simulink model "ADCS_Software_v1"  (R2026a)
settings: Solver=FixedStepAuto  StopTime=Inf  FixedStep=0.05  MaxStep=0.1
model workspace (MAT data in the model file):
  I_RW = Simulink.Parameter
  I_RW.Value = 1
  I_RW.Complexity = 'real'
  I_RW.Dimensions = [1 1]
  I_RW.CoderInfo.StorageClass = 'ExportedGlobal'
  I_RW.DataType = 'auto'
  Sig = Simulink.Signal
  Sig.Dimensions = -1
  Sig.DimensionsMode = 'auto'
  Sig.Complexity = 'auto'
  Sig.SampleTime = -1
  Sig.SamplingMode = 'auto'
  Sig.DataType = 'auto'
  h_max = Simulink.Parameter
  h_max.Value = 1.47
  h_max.Complexity = 'real'
  h_max.Dimensions = [1 1]
  h_max.DataType = 'auto'
  k_desat = Simulink.Parameter
  k_desat.Value = 1
  k_desat.Complexity = 'real'
  k_desat.Dimensions = [1 1]
  k_desat.CoderInfo.StorageClass = 'ExportedGlobal'
  k_desat.DataType = 'auto'
  kd_detumble = Simulink.Parameter
  kd_detumble.Value = 1
  kd_detumble.Complexity = 'real'
  kd_detumble.Dimensions = [1 1]
  kd_detumble.CoderInfo.StorageClass = 'ExportedGlobal'
  kd_detumble.DataType = 'auto'
  kd_hold = Simulink.Parameter
  kd_hold.Value = 1
  kd_hold.Complexity = 'real'
  kd_hold.Dimensions = [1 1]
  kd_hold.CoderInfo.StorageClass = 'ExportedGlobal'
  kd_hold.DataType = 'auto'
  kd_point = Simulink.Parameter
  kd_point.Value = 20
  kd_point.Complexity = 'real'
  kd_point.Dimensions = [1 1]
  kd_point.CoderInfo.StorageClass = 'ExportedGlobal'
  kd_point.DataType = 'auto'
  kd_slew_fast = Simulink.Parameter
  kd_slew_fast.Value = 1
  kd_slew_fast.Complexity = 'real'
  kd_slew_fast.Dimensions = [1 1]
  kd_slew_fast.CoderInfo.StorageClass = 'ExportedGlobal'
  kd_slew_fast.DataType = 'auto'
  kd_slew_slow = Simulink.Parameter
  kd_slew_slow.Value = 1
  kd_slew_slow.Complexity = 'real'
  kd_slew_slow.Dimensions = [1 1]
  kd_slew_slow.CoderInfo.StorageClass = 'ExportedGlobal'
  kd_slew_slow.DataType = 'auto'
  kd_spin = Simulink.Parameter
  kd_spin.Value = 0
  kd_spin.Complexity = 'real'
  kd_spin.Dimensions = [1 1]
  kd_spin.CoderInfo.StorageClass = 'ExportedGlobal'
  kd_spin.DataType = 'auto'
  kp_hold = Simulink.Parameter
  kp_hold.Value = 1
  kp_hold.Complexity = 'real'
  kp_hold.Dimensions = [1 1]
  kp_hold.CoderInfo.StorageClass = 'ExportedGlobal'
  kp_hold.DataType = 'auto'
  kp_point = Simulink.Parameter
  kp_point.Value = 2
  kp_point.Complexity = 'real'
  kp_point.Dimensions = [1 1]
  kp_point.CoderInfo.StorageClass = 'ExportedGlobal'
  kp_point.DataType = 'auto'
  kp_slew_fast = Simulink.Parameter
  kp_slew_fast.Value = 1
  kp_slew_fast.Complexity = 'real'
  kp_slew_fast.Dimensions = [1 1]
  kp_slew_fast.CoderInfo.StorageClass = 'ExportedGlobal'
  kp_slew_fast.DataType = 'auto'
  kp_slew_slow = Simulink.Parameter
  kp_slew_slow.Value = 1
  kp_slew_slow.Complexity = 'real'
  kp_slew_slow.Dimensions = [1 1]
  kp_slew_slow.CoderInfo.StorageClass = 'ExportedGlobal'
  kp_slew_slow.DataType = 'auto'
  kp_spin = Simulink.Parameter
  kp_spin.Value = 1
  kp_spin.Complexity = 'real'
  kp_spin.Dimensions = [1 1]
  kp_spin.CoderInfo.StorageClass = 'ExportedGlobal'
  kp_spin.DataType = 'auto'
values from neighbouring files (symbols this model uses):
  h_max = 1.47    [parameters.m]
  I_RW = 1    [parameters.m]
  k_desat = 1    [parameters.m]
  kd_detumble = 1    [parameters.m]
  kd_point = 20    [parameters.m]
  kd_spin = 0    [parameters.m]
  kp_point = 2    [parameters.m]
  kp_spin = 1    [parameters.m]
  omega_thr = 0.1    [parameters.m]
  omega_zero = 0.01    [parameters.m]
libraries: matrix_library x10, simulink x4, aerolibutil x2
(part 1 of 2)
settings Model: Creator=ADMIN  LastModifiedBy=Administrator
settings DataIOCC: ExternalInput=ds
settings RTWCC: GenerateReport=on  LaunchReport=on
settings SimscapeCC: SimscapeNominalValues="[{\"value\":\"1\",\"unit\":\"A\"},{\"value\":\"1\",\"unit\":\"bar\"},{\"value\":\"1\",\"unit\":\"cm^2\"},{\"value\":\"1\",\"unit\":\"cm^3/s\"},{\"value\":\"1\",\"unit\":\"kJ/kg\"},{\"value\":\"1\",\"unit\":\"kW\"},{\"value\":\"1\",\"unit\":\"l\"},{\"value\":\"1\",\"unit\":\"N\"},{\"value\":\"1\",\"unit\":\"N*m\"},{\"value\":\"1\",\"unit\":\"V\"}]"  SimscapeLogType=none  SimscapeLogDataHistory=5000.0

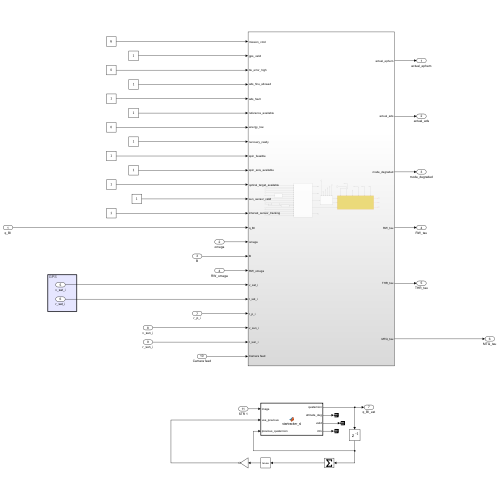
[thumbnail: Simulink's stored preview of the top-level diagram]
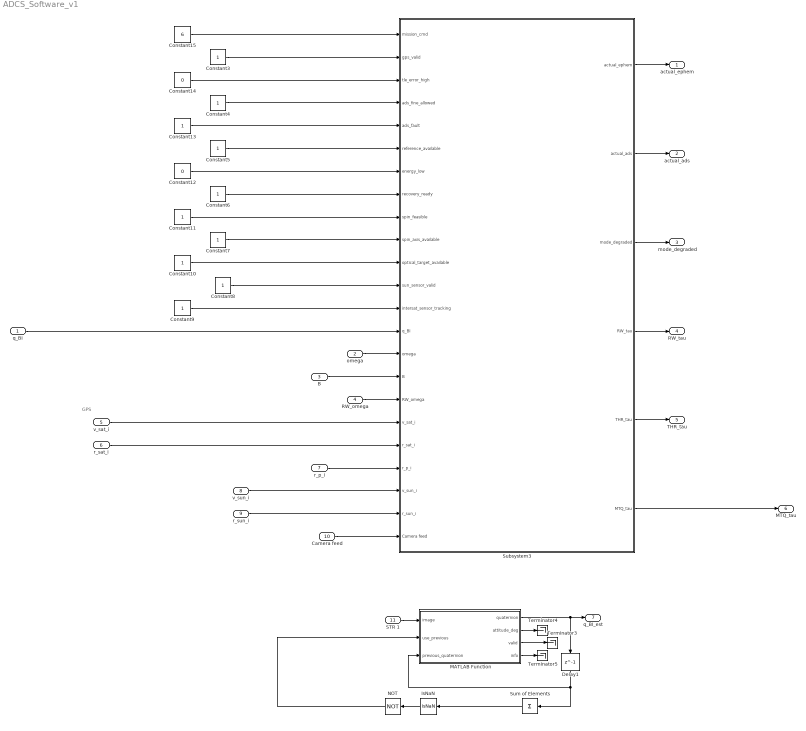
== system ADCS_Software_v1 ==
  note: GPS
  q_BI : Inport
  omega : Inport  Port=2
  B : Inport  Port=3
  RW_omega : Inport  Port=4
  v_sat_i : Inport  Port=5
  r_sat_i : Inport  Port=6
  r_p_i : Inport  Port=7
  v_sun_i : Inport  Port=8  OutDataTypeStr=double  PortDimensions=3
  r_sun_i : Inport  Port=9  OutDataTypeStr=double  PortDimensions=3
  Camera feed : Inport  Port=10  OutDataTypeStr=uint8  PortDimensions=[512,512]
  STR 1 : Inport  Port=11  OutDataTypeStr=uint8  PortDimensions=[1024,1024]
  Constant{3..11,13} (10 alike) : Constant  OutDataTypeStr=boolean
  Constant12 : Constant  Value=0  OutDataTypeStr=boolean
  Constant14 : Constant  Value=0  OutDataTypeStr=boolean
  Constant15 : Constant  Value=6  OutDataTypeStr=uint8
  Delay1 : Delay  DelayLength=1  InitialCondition=nan
  IsNaN : RelationalOperator  Operator=isNaN  OutDataTypeStr=boolean  RndMeth=Simplest  InputSameDT=off
  MATLAB Function : MATLAB Function  TreatAsAtomicUnit=on
  NOT : Logic  Operator=NOT  IconShape=distinctive  AllPortsSameDT=off  OutDataTypeStr=boolean
  Subsystem3 : Subsystem
  Sum of Elements : Sum  Inputs=+
  Terminator3 : Terminator
  Terminator4 : Terminator
  Terminator5 : Terminator
  actual_ephem : Outport
  actual_ads : Outport  Port=2
  mode_degraded : Outport  Port=3
  RW_tau : Outport  Port=4
  THR_tau : Outport  Port=5
  MTQ_tau : Outport  Port=6
  q_BI_est : Outport  Port=7  PortDimensions=[1 4]
  wires:
  Constant13/1 -> Subsystem3/5(ads_fault)
  Constant3/1 -> Subsystem3/2(gps_valid)
  Constant15/1 -> Subsystem3/1(mission_cmd)
  Constant14/1 -> Subsystem3/3(tle_error_high)
  Constant4/1 -> Subsystem3/4(ads_fine_allowed)
  Constant5/1 -> Subsystem3/6(reference_available)
  Constant12/1 -> Subsystem3/7(energy_low)
  Constant6/1 -> Subsystem3/8(recovery_ready)
  Constant10/1 -> Subsystem3/11(optical_target_available)
  Constant7/1 -> Subsystem3/10(spin_axis_available)
  Constant11/1 -> Subsystem3/9(spin_feasible)
  Constant8/1 -> Subsystem3/12(sun_sensor_valid)
  Constant9/1 -> Subsystem3/13(intersat_sensor_tracking)
  Subsystem3/1(actual_ephem) -> actual_ephem/1
  Subsystem3/2(actual_ads) -> actual_ads/1
  Subsystem3/3(mode_degraded) -> mode_degraded/1
  Subsystem3/4(RW_tau) -> RW_tau/1
  Subsystem3/5(THR_tau) -> THR_tau/1
  Subsystem3/6(MTQ_tau) -> MTQ_tau/1
  omega/1 -> Subsystem3/15(omega)
  B/1 -> Subsystem3/16(B)
  RW_omega/1 -> Subsystem3/17(RW_omega)
  v_sat_i/1 -> Subsystem3/18(v_sat_i)
  r_sat_i/1 -> Subsystem3/19(r_sat_i)
  r_p_i/1 -> Subsystem3/20(r_p_i)
  v_sun_i/1 -> Subsystem3/21(v_sun_i)
  r_sun_i/1 -> Subsystem3/22(r_sun_i)
  Camera feed/1 -> Subsystem3/23(Camera feed)
  q_BI/1 -> Subsystem3/14(q_BI)
  STR 1/1 -> MATLAB Function/1(image)
  MATLAB Function/1(quaternion) -> q_BI_est/1, Delay1/1
  MATLAB Function/4(info) -> Terminator5/1
  MATLAB Function/3(valid) -> Terminator3/1
  MATLAB Function/2(attitude_deg) -> Terminator4/1
  Sum of Elements/1 -> IsNaN/1
  IsNaN/1 -> NOT/1
  NOT/1 -> MATLAB Function/2(use_previous)
  Delay1/1 -> MATLAB Function/3(previous_quaternion), Sum of Elements/1

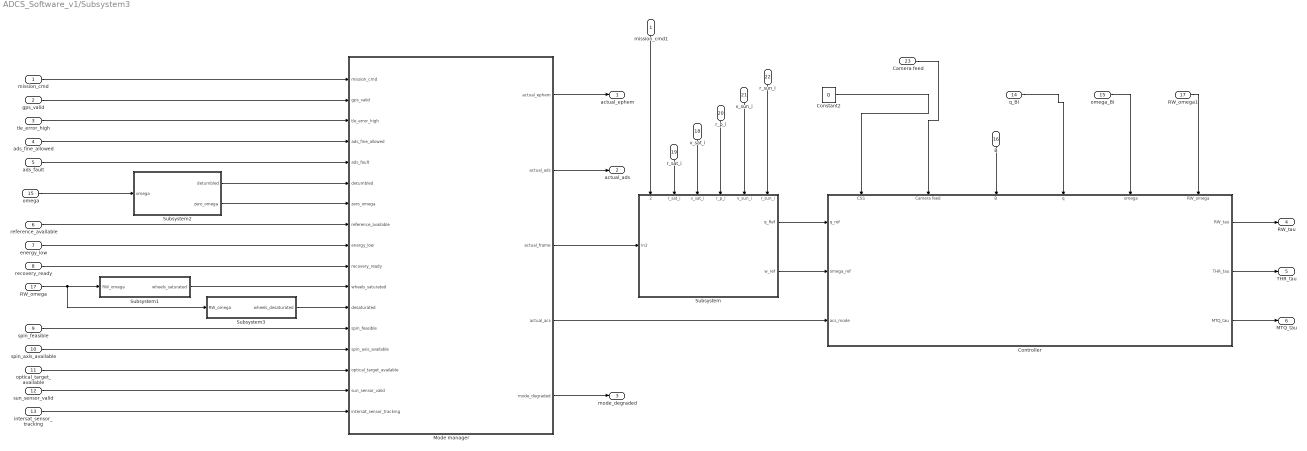
== system ADCS_Software_v1/Subsystem3 ==
  mission_cmd : Inport
  gps_valid : Inport  Port=2
  tle_error_high : Inport  Port=3
  ads_fine_allowed : Inport  Port=4
  ads_fault : Inport  Port=5
  reference_available : Inport  Port=6
  energy_low : Inport  Port=7
  recovery_ready : Inport  Port=8
  spin_feasible : Inport  Port=9
  spin_axis_available : Inport  Port=10
  optical_target_available : Inport  Port=11
  sun_sensor_valid : Inport  Port=12
  intersat_sensor_tracking : Inport  Port=13
  q_BI : Inport  Port=14
  omega : Inport  Port=15
  B : Inport  Port=16
  RW_omega : Inport  Port=17
  v_sat_i : Inport  Port=18
  r_sat_i : Inport  Port=19
  r_p_i : Inport  Port=20
  v_sun_i : Inport  Port=21
  r_sun_i : Inport  Port=22
  Camera feed : Inport  Port=23
  Constant2 : Constant  Value=0
  Controller : Subsystem
      settings: PortSchema="{\"entries\":[{\"content\":{\"sides\":[{\"content\":{\"connectorIds\":[\"In1\",\"In2\",\"In3\"]},\"type\":\"ConnectorPlacement.EquallySpacedRectSide\",\"uuid\":\"3d0ce77c-a0dd-4e63-bb58-aa259872b360\"},{\"content\":{\"connectorIds\":[\"Out1\",\"Out2\",\"Out3\"],\"side\":\"RIGHT\"},\"type\":\"ConnectorPlacement.EquallySpacedRectSide\",\"uuid\":\"c51ce6d0-00d2-499a-9be1-102c03c9909c\"},{\"content\":{\"connectorIds\":[\"In4\",\"In5\",\"In6\",\"In7\",\"In8\",\"In9\"],\"side\":\"TOP\"},\"type\":\"ConnectorPlacement.EquallySpacedRectSide\",\"uuid\":\"ed1e7bc4-2cca-4611-893f-1128994bf2d9\"},{\"content\":{\"side\":\"BOTTOM\"},\"type\":\"ConnectorPlacement.EquallySpacedRectSide\",\"uuid\":\"574e7f6a-1005-4b0c-82f8-22f1ef6841a8\"}]},\"type\":\"ConnectorPlacement.EquallySpacedConnector\",\"uuid\":\"15c446ec-b512-4968-b865-507fd68d8b0b\"}],\"packageUris\":[\"http://schema.mathworks.com/mf0/Connector/R2020b\"],\"version\":\"1.0\"}"
  Mode manager : Subsystem
  RW_omega1 : InportShadow  Port=17
  Subsystem : Subsystem
      settings: PortSchema="{\"entries\":[{\"content\":{\"sides\":[{\"content\":{\"connectorIds\":[\"In1\"]},\"type\":\"ConnectorPlacement.EquallySpacedRectSide\",\"uuid\":\"74bf1b15-53db-441c-9152-7c9ad8598452\"},{\"content\":{\"connectorIds\":[\"Out1\",\"Out2\"],\"side\":\"RIGHT\"},\"type\":\"ConnectorPlacement.EquallySpacedRectSide\",\"uuid\":\"e98e0885-3f20-4aa1-b3a1-f2c890def05c\"},{\"content\":{\"connectorIds\":[\"In2\",\"In3\",\"In4\",\"In5\",\"In6\",\"In7\"],\"side\":\"TOP\"},\"type\":\"ConnectorPlacement.EquallySpacedRectSide\",\"uuid\":\"f0898a47-7ae2-48e7-af8a-6d6327a5175a\"}]},\"type\":\"ConnectorPlacement.EquallySpacedConnector\",\"uuid\":\"b563a257-d36a-4c1e-a9df-51a9ac9caccd\"}],\"packageUris\":[\"http://schema.mathworks.com/mf0/Connector/R2020b\"],\"version\":\"1.0\"}"
  Subsystem1 : Subsystem
  Subsystem2 : Subsystem
  Subsystem3 : Subsystem
  mission_cmd1 : InportShadow
  omega_BI : InportShadow  Port=15
  actual_ephem : Outport
  actual_ads : Outport  Port=2
  mode_degraded : Outport  Port=3
  RW_tau : Outport  Port=4
  THR_tau : Outport  Port=5
  MTQ_tau : Outport  Port=6
  wires:
  spin_axis_available/1 -> Mode manager/14(spin_axis_available)
  Controller/1(RW_tau) -> RW_tau/1
  Mode manager/1(actual_ephem) -> actual_ephem/1
  Mode manager/5(mode_degraded) -> mode_degraded/1
  Constant2/1 -> Controller/4(CSS)
  gps_valid/1 -> Mode manager/2(gps_valid)
  RW_omega/1 -> Subsystem3/1(RW_omega), Subsystem1/1(RW_omega)
  Subsystem2/1(detumbled) -> Mode manager/6(detumbled)
  Mode manager/2(actual_ads) -> actual_ads/1
  tle_error_high/1 -> Mode manager/3(tle_error_high)
  Controller/3(MTQ_tau) -> MTQ_tau/1
  Mode manager/4(actual_acs) -> Controller/3(acs_mode)
  Subsystem1/1(wheels_saturated) -> Mode manager/11(wheels_saturated)
  sun_sensor_valid/1 -> Mode manager/16(sun_sensor_valid)
  recovery_ready/1 -> Mode manager/10(recovery_ready)
  Subsystem3/1(wheels_desaturated) -> Mode manager/12(desaturated)
  ads_fine_allowed/1 -> Mode manager/4(ads_fine_allowed)
  spin_feasible/1 -> Mode manager/13(spin_feasible)
  ads_fault/1 -> Mode manager/5(ads_fault)
  energy_low/1 -> Mode manager/9(energy_low)
  intersat_sensor_tracking/1 -> Mode manager/17(intersat_sensor_tracking)
  optical_target_available/1 -> Mode manager/15(optical_target_available)
  mission_cmd/1 -> Mode manager/1(mission_cmd)
  omega/1 -> Subsystem2/1(omega)
  reference_available/1 -> Mode manager/8(reference_available)
  Controller/2(THR_tau) -> THR_tau/1
  RW_omega1/1 -> Controller/9(RW_omega)
  omega_BI/1 -> Controller/8(omega)
  B/1 -> Controller/6(B)
  Mode manager/3(actual_frame) -> Subsystem/1(In2)
  Subsystem/1(q_Ref) -> Controller/1(q_ref)
  Subsystem/2(w_ref) -> Controller/2(omega_ref)
  v_sat_i/1 -> Subsystem/4(v_sat_i)
  r_sat_i/1 -> Subsystem/3(r_sat_i)
  r_p_i/1 -> Subsystem/5(r_p_i)
  v_sun_i/1 -> Subsystem/6(v_sun_i)
  r_sun_i/1 -> Subsystem/7(r_sun_i)
  Subsystem2/2(zero_omega) -> Mode manager/7(zero_omega)
  q_BI/1 -> Controller/7(q)
  Camera feed/1 -> Controller/5(Camera feed)
  mission_cmd1/1 -> Subsystem/2(mission_cmd)

== system ADCS_Software_v1/Subsystem3/Controller ==
  q_ref : Inport
  omega_ref : Inport  Port=2
  acs_mode : Inport  Port=3
  CSS : Inport  Port=4
  Camera feed : Inport  Port=5
  B : Inport  Port=6
  q : Inport  Port=7
  omega : Inport  Port=8
  RW_omega : Inport  Port=9
  Control Algorithms : Subsystem
  "error " : Subsystem
  omega1 : InportShadow  Port=8
  RW_tau : Outport
  THR_tau : Outport  Port=2
  MTQ_tau : Outport  Port=3
  wires:
  "error "/1(q_err) -> Control Algorithms/7(q_err)
  RW_omega/1 -> Control Algorithms/4(RW_omega)
  CSS/1 -> Control Algorithms/2(CSS)
  Camera feed/1 -> Control Algorithms/5(Camera feed)
  omega/1 -> Control Algorithms/3(omega)
  B/1 -> Control Algorithms/6(B)
  "error "/2(omega_err) -> Control Algorithms/8(omega_err)
  Control Algorithms/1(THR_tau) -> THR_tau/1
  Control Algorithms/2(MTQ_tau) -> MTQ_tau/1
  Control Algorithms/3(RW_tau) -> RW_tau/1
  q_ref/1 -> "error "/1(q_ref)
  q/1 -> "error "/2(q_BI)
  omega_ref/1 -> "error "/3(omega_ref)
  omega1/1 -> "error "/4(omega)
  acs_mode/1 -> Control Algorithms/1(acs_mode)

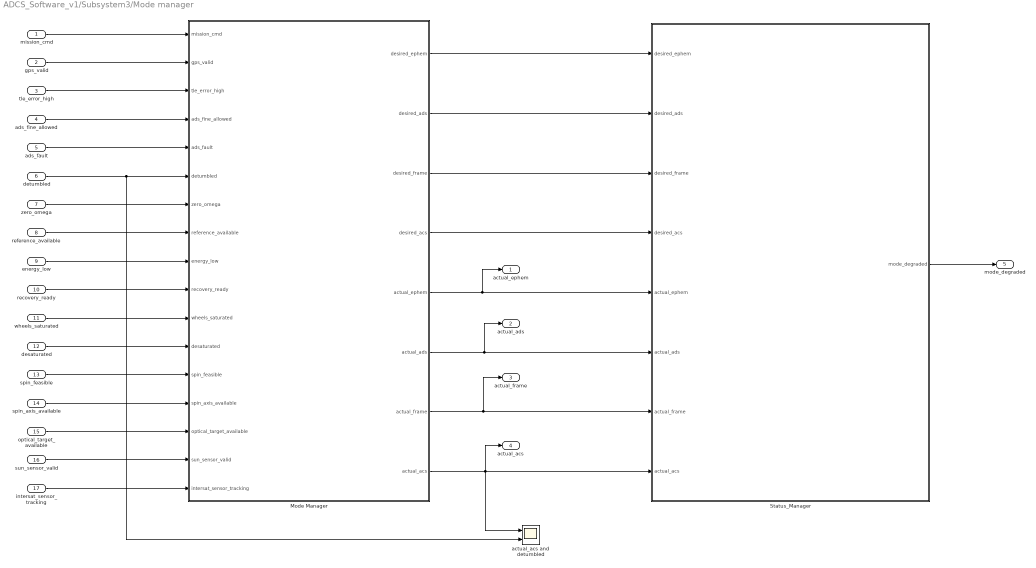
== system ADCS_Software_v1/Subsystem3/Mode manager ==
  mission_cmd : Inport
  gps_valid : Inport  Port=2
  tle_error_high : Inport  Port=3
  ads_fine_allowed : Inport  Port=4
  ads_fault : Inport  Port=5
  detumbled : Inport  Port=6
  zero_omega : Inport  Port=7
  reference_available : Inport  Port=8
  energy_low : Inport  Port=9
  recovery_ready : Inport  Port=10
  wheels_saturated : Inport  Port=11
  desaturated : Inport  Port=12
  spin_feasible : Inport  Port=13
  spin_axis_available : Inport  Port=14
  optical_target_available : Inport  Port=15
  sun_sensor_valid : Inport  Port=16
  intersat_sensor_tracking : Inport  Port=17
  Mode Manager : Subsystem
  Status_Manager : Stateflow chart  TreatAsAtomicUnit=on
  actual_acs and detumbled : Scope  NumInputPorts=2
      settings: ActiveDisplayYMinimum=-0.74999999999999978  ActiveDisplayYMaximum=6.75  DataLoggingVariableName=ScopeData3
  actual_ephem : Outport
  actual_ads : Outport  Port=2
  actual_frame : Outport  Port=3
  actual_acs : Outport  Port=4
  mode_degraded : Outport  Port=5
  wires:
  recovery_ready/1 -> Mode Manager/10(recovery_ready)
  Mode Manager/2(desired_ads) -> Status_Manager/2(desired_ads)
  Mode Manager/8(actual_acs) -> actual_acs/1, Status_Manager/8(actual_acs), actual_acs and detumbled/1
  Mode Manager/1(desired_ephem) -> Status_Manager/1(desired_ephem)
  Mode Manager/5(actual_ephem) -> actual_ephem/1, Status_Manager/5(actual_ephem)
  Mode Manager/6(actual_ads) -> actual_ads/1, Status_Manager/6(actual_ads)
  Mode Manager/7(actual_frame) -> actual_frame/1, Status_Manager/7(actual_frame)
  Mode Manager/3(desired_frame) -> Status_Manager/3(desired_frame)
  Mode Manager/4(desired_acs) -> Status_Manager/4(desired_acs)
  reference_available/1 -> Mode Manager/8(reference_available)
  mission_cmd/1 -> Mode Manager/1(mission_cmd)
  ads_fault/1 -> Mode Manager/5(ads_fault)
  ads_fine_allowed/1 -> Mode Manager/4(ads_fine_allowed)
  wheels_saturated/1 -> Mode Manager/11(wheels_saturated)
  optical_target_available/1 -> Mode Manager/15(optical_target_available)
  detumbled/1 -> Mode Manager/6(detumbled), actual_acs and detumbled/2
  intersat_sensor_tracking/1 -> Mode Manager/17(intersat_sensor_tracking)
  desaturated/1 -> Mode Manager/12(desaturated)
  spin_feasible/1 -> Mode Manager/13(spin_feasible)
  tle_error_high/1 -> Mode Manager/3(tle_error_high)
  energy_low/1 -> Mode Manager/9(energy_low)
  Status_Manager/1(mode_degraded) -> mode_degraded/1
  spin_axis_available/1 -> Mode Manager/14(spin_axis_available)
  sun_sensor_valid/1 -> Mode Manager/16(sun_sensor_valid)
  gps_valid/1 -> Mode Manager/2(gps_valid)
  zero_omega/1 -> Mode Manager/7(zero_omega)

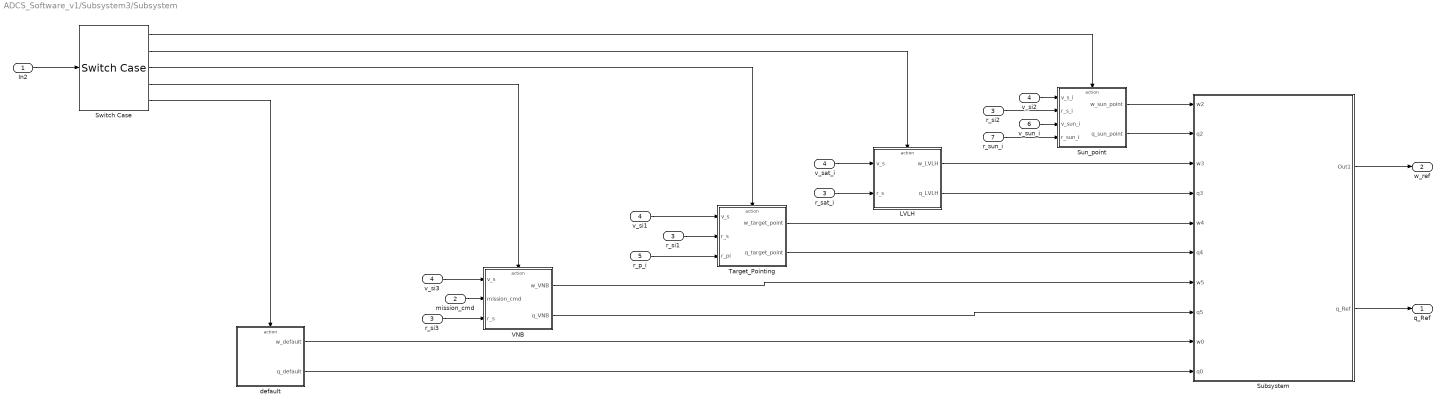
== system ADCS_Software_v1/Subsystem3/Subsystem ==
  In2 : Inport
  mission_cmd : Inport  Port=2
  r_sat_i : Inport  Port=3
  v_sat_i : Inport  Port=4
  r_p_i : Inport  Port=5
  v_sun_i : Inport  Port=6
  r_sun_i : Inport  Port=7
  LVLH : Subsystem
  Subsystem : Subsystem
  Sun_point : Subsystem
  Switch Case : SwitchCase  CaseConditions={2,3,4,5}
  Target_Pointing : Subsystem
  VNB : Subsystem
  default : Subsystem
  r_si1 : InportShadow  Port=3
  r_si2 : InportShadow  Port=3
  r_si3 : InportShadow  Port=3
  v_si1 : InportShadow  Port=4
  v_si2 : InportShadow  Port=4
  v_si3 : InportShadow  Port=4
  q_Ref : Outport
  w_ref : Outport  Port=2
  wires:
  Switch Case/5 -> default/Action
  In2/1 -> Switch Case/1
  r_si1/1 -> Target_Pointing/2(r_s)
  v_si1/1 -> Target_Pointing/1(v_s)
  LVLH/1(w_LVLH) -> Subsystem/3(w3)
  LVLH/2(q_LVLH) -> Subsystem/4(q3)
  Target_Pointing/1(w_target_point) -> Subsystem/5(w4)
  Target_Pointing/2(q_target_point) -> Subsystem/6(q4)
  default/1(w_default) -> Subsystem/9(w0)
  default/2(q_default) -> Subsystem/10(q0)
  Subsystem/1(Out1) -> w_ref/1
  v_sat_i/1 -> LVLH/1(v_s)
  r_sat_i/1 -> LVLH/2(r_s)
  v_si2/1 -> Sun_point/1(v_s_i)
  r_si2/1 -> Sun_point/2(r_s_i)
  Sun_point/1(w_sun_point) -> Subsystem/1(w2)
  Sun_point/2(q_sun_point) -> Subsystem/2(q2)
  r_p_i/1 -> Target_Pointing/3(r_pi)
  v_sun_i/1 -> Sun_point/3(v_sun_i)
  r_sun_i/1 -> Sun_point/4(r_sun_i)
  Switch Case/1 -> Sun_point/Action
  Switch Case/2 -> LVLH/Action
  Switch Case/3 -> Target_Pointing/Action
  Subsystem/2(q_Ref) -> q_Ref/1
  r_si3/1 -> VNB/3(r_s)
  v_si3/1 -> VNB/1(v_s)
  VNB/2(q_VNB) -> Subsystem/8(q5)
  VNB/1(w_VNB) -> Subsystem/7(w5)
  Switch Case/4 -> VNB/Action
  mission_cmd/1 -> VNB/2(mission_cmd)

== system ADCS_Software_v1/Subsystem3/Subsystem1 ==
  RW_omega : Inport
  Abs : Abs  SaturateOnIntegerOverflow=off
  Compare To Constant : simulink/Logic and Bit Operations/Compare To Constant  relop=>=  const=h_max*0.95  OutDataTypeStr=boolean
  Gain : Gain  Gain=I_RW
  Max of Elements : MinMax  Function=max
  wheels_saturated : Outport
  wires:
  Gain/1 -> Compare To Constant/1
  Abs/1 -> Max of Elements/1
  RW_omega/1 -> Abs/1
  Max of Elements/1 -> Gain/1
  Compare To Constant/1 -> wheels_saturated/1

== system ADCS_Software_v1/Subsystem3/Subsystem2 ==
  omega : Inport
  Compare To Constant : simulink/Logic and Bit Operations/Compare To Constant  relop=<=  const=omega_thr^2  OutDataTypeStr=boolean
  Compare To Constant1 : simulink/Logic and Bit Operations/Compare To Constant  relop=<=  const=omega_zero^2  OutDataTypeStr=boolean
  Dot Product : DotProduct  OutDataTypeStr=Inherit: Inherit via internal rule
  detumbled : Outport
  zero_omega : Outport  Port=2
  wires:
  Compare To Constant/1 -> detumbled/1
  omega/1 -> Dot Product/2, Dot Product/1
  Dot Product/1 -> Compare To Constant1/1, Compare To Constant/1
  Compare To Constant1/1 -> zero_omega/1

== system ADCS_Software_v1/Subsystem3/Subsystem3 ==
  RW_omega : Inport
  Abs : Abs  SaturateOnIntegerOverflow=off
  Compare To Constant : simulink/Logic and Bit Operations/Compare To Constant  relop=<=  const=h_max*0.25  OutDataTypeStr=boolean
  Gain : Gain  Gain=I_RW
  Max of Elements : MinMax  Function=max
  wheels_desaturated : Outport
  wires:
  Compare To Constant/1 -> wheels_desaturated/1
  Max of Elements/1 -> Gain/1
  RW_omega/1 -> Abs/1
  Abs/1 -> Max of Elements/1
  Gain/1 -> Compare To Constant/1

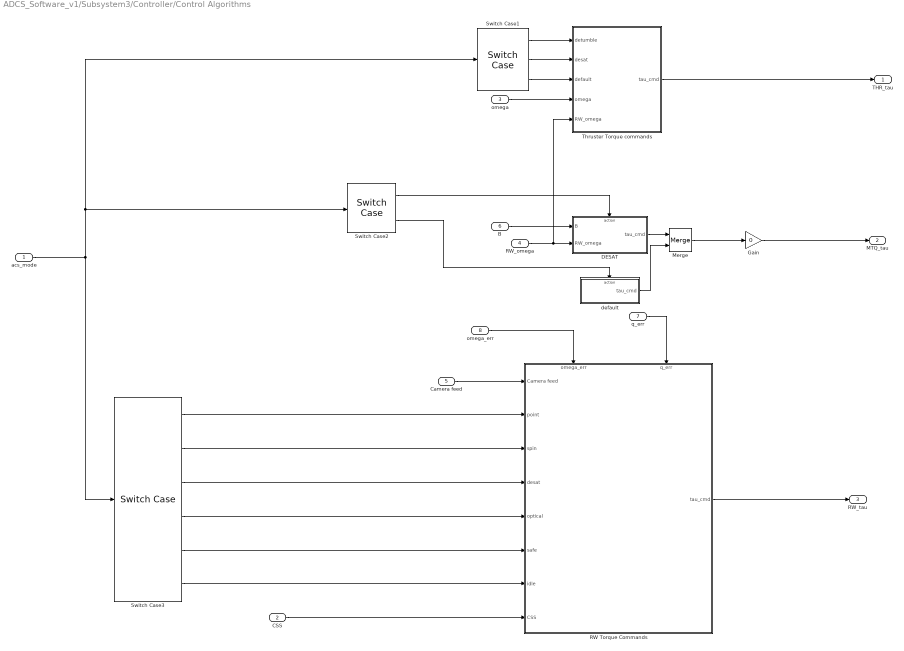
== system ADCS_Software_v1/Subsystem3/Controller/Control Algorithms ==
  acs_mode : Inport
  CSS : Inport  Port=2
  omega : Inport  Port=3
  RW_omega : Inport  Port=4
  Camera feed : Inport  Port=5
  B : Inport  Port=6
  q_err : Inport  Port=7
  omega_err : Inport  Port=8
  DESAT : Subsystem  TreatAsAtomicUnit=on
  Gain : Gain  Gain=0
  Merge : Merge
  RW Torque Commands : Subsystem
      settings: PortSchema="{\"entries\":[{\"content\":{\"sides\":[{\"content\":{\"connectorIds\":[\"In1\",\"In2\",\"In3\",\"In4\",\"In5\",\"In6\",\"In7\",\"In8\"]},\"type\":\"ConnectorPlacement.EquallySpacedRectSide\",\"uuid\":\"3d0ce77c-a0dd-4e63-bb58-aa259872b360\"},{\"content\":{\"connectorIds\":[\"Out1\"],\"side\":\"RIGHT\"},\"type\":\"ConnectorPlacement.EquallySpacedRectSide\",\"uuid\":\"c51ce6d0-00d2-499a-9be1-102c03c9909c\"},{\"content\":{\"connectorIds\":[\"In9\",\"In10\"],\"side\":\"TOP\"},\"type\":\"ConnectorPlacement.EquallySpacedRectSide\",\"uuid\":\"ed1e7bc4-2cca-4611-893f-1128994bf2d9\"}]},\"type\":\"ConnectorPlacement.EquallySpacedConnector\",\"uuid\":\"15c446ec-b512-4968-b865-507fd68d8b0b\"}],\"packageUris\":[\"http://schema.mathworks.com/mf0/Connector/R2020b\"],\"version\":\"1.0\"}"
  Switch Case1 : SwitchCase  CaseConditions={1,4}
  Switch Case2 : SwitchCase  CaseConditions={4}
  Switch Case3 : SwitchCase  CaseConditions={2,3,4,5,6}
  Thruster Torque commands : Subsystem
  default : Subsystem  TreatAsAtomicUnit=on
  THR_tau : Outport
  MTQ_tau : Outport  Port=2
  RW_tau : Outport  Port=3
  wires:
  Camera feed/1 -> RW Torque Commands/1(Camera feed)
  RW_omega/1 -> Thruster Torque commands/5(RW_omega), DESAT/2(RW_omega)
  B/1 -> DESAT/1(B)
  CSS/1 -> RW Torque Commands/8(CSS)
  omega/1 -> Thruster Torque commands/4(omega)
  omega_err/1 -> RW Torque Commands/9(omega_err)
  q_err/1 -> RW Torque Commands/10(q_err)
  Switch Case1/1 -> Thruster Torque commands/1(detumble)
  Switch Case1/3 -> Thruster Torque commands/3(default)
  default/1(tau_cmd) -> Merge/2
  Switch Case2/2 -> default/Action
  DESAT/1(tau_cmd) -> Merge/1
  Merge/1 -> Gain/1
  Switch Case2/1 -> DESAT/Action
  Switch Case3/1 -> RW Torque Commands/2(point)
  Switch Case3/2 -> RW Torque Commands/3(spin)
  Switch Case3/3 -> RW Torque Commands/4(desat)
  Switch Case3/6 -> RW Torque Commands/7(idle)
  acs_mode/1 -> Switch Case3/1, Switch Case1/1, Switch Case2/1
  Gain/1 -> MTQ_tau/1
  RW Torque Commands/1(tau_cmd) -> RW_tau/1
  Thruster Torque commands/1(tau_cmd) -> THR_tau/1
  Switch Case1/2 -> Thruster Torque commands/2(desat)
  Switch Case3/4 -> RW Torque Commands/5(optical)
  Switch Case3/5 -> RW Torque Commands/6(safe)

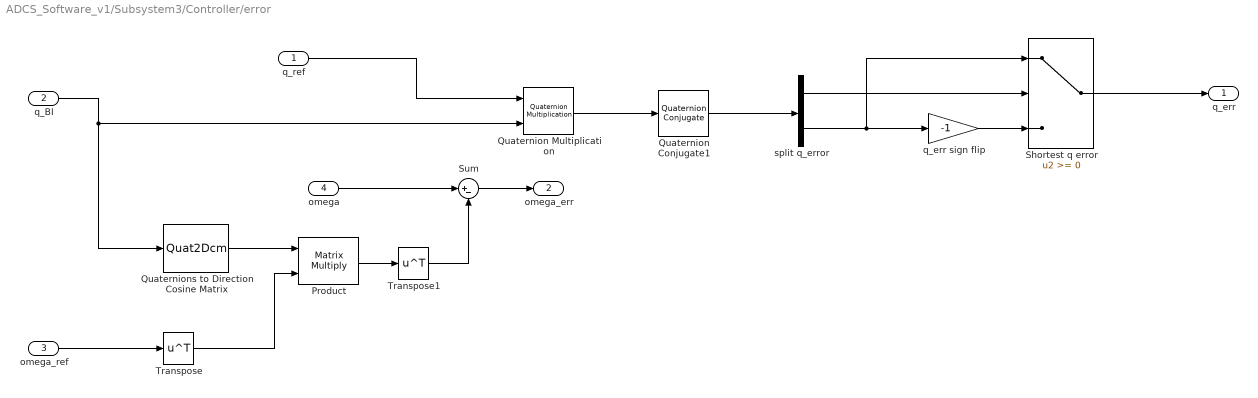
== system ADCS_Software_v1/Subsystem3/Controller/error  ==
  q_ref : Inport
  q_BI : Inport  Port=2
  omega_ref : Inport  Port=3
  omega : Inport  Port=4
  Product : Product  Multiplication=Matrix(*)
  Quaternion Conjugate1 : aerolibutil/Quaternion Conjugate
  Quaternion Multiplication : aerolibutil/Quaternion Multiplication
  Quaternions to Direction Cosine Matrix : Quat2Dcm
  Shortest q error : Switch  SaturateOnIntegerOverflow=off  InputSameDT=off
  Sum : Sum  Inputs=|+-
  Transpose : Math  Operator=transpose
  Transpose1 : Math  Operator=transpose
  q_err sign flip : Gain  Gain=-1
  split q_error : Demux  Outputs=[1 3]
  q_err : Outport
  omega_err : Outport  Port=2
  wires:
  Sum/1 -> omega_err/1
  Quaternion Multiplication/1 -> Quaternion Conjugate1/1
  q_BI/1 -> Quaternions to Direction Cosine Matrix/1, Quaternion Multiplication/2
  omega/1 -> Sum/1
  Shortest q error/1 -> q_err/1
  split q_error/2 -> Shortest q error/1, q_err sign flip/1
  split q_error/1 -> Shortest q error/2
  q_err sign flip/1 -> Shortest q error/3
  Quaternions to Direction Cosine Matrix/1 -> Product/1
  Product/1 -> Transpose1/1
  omega_ref/1 -> Transpose/1
  Transpose/1 -> Product/2
  Transpose1/1 -> Sum/2
  Quaternion Conjugate1/1 -> split q_error/1
  q_ref/1 -> Quaternion Multiplication/1

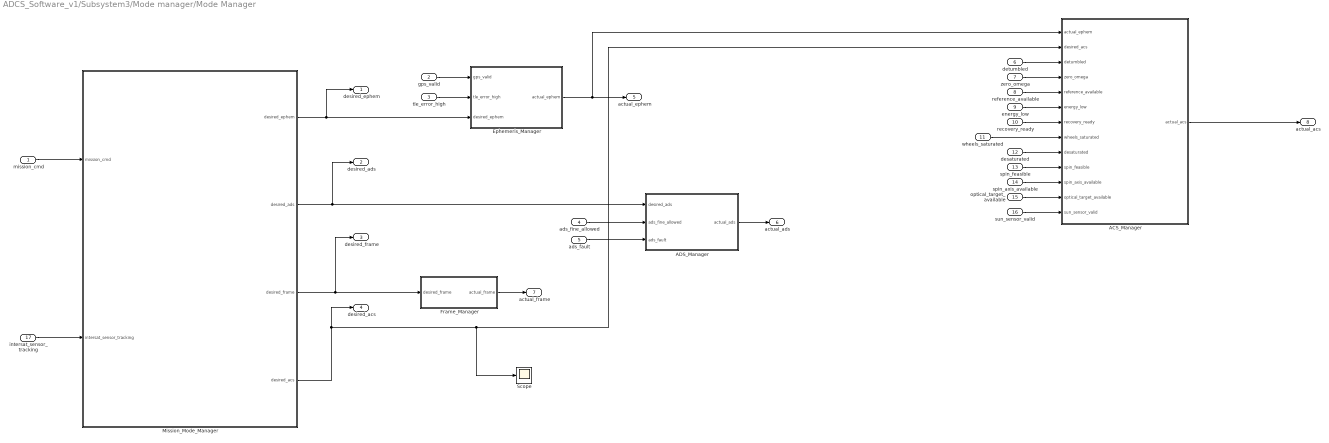
== system ADCS_Software_v1/Subsystem3/Mode manager/Mode Manager ==
  mission_cmd : Inport  OutDataTypeStr=uint8  PortDimensions=1
  gps_valid : Inport  Port=2  OutDataTypeStr=boolean  PortDimensions=1
  tle_error_high : Inport  Port=3  OutDataTypeStr=boolean  PortDimensions=1
  ads_fine_allowed : Inport  Port=4  OutDataTypeStr=boolean  PortDimensions=1
  ads_fault : Inport  Port=5  OutDataTypeStr=boolean  PortDimensions=1
  detumbled : Inport  Port=6  OutDataTypeStr=boolean  PortDimensions=1
  zero_omega : Inport  Port=7
  reference_available : Inport  Port=8  OutDataTypeStr=boolean  PortDimensions=1
  energy_low : Inport  Port=9  OutDataTypeStr=boolean  PortDimensions=1
  recovery_ready : Inport  Port=10  OutDataTypeStr=boolean  PortDimensions=1
  wheels_saturated : Inport  Port=11  OutDataTypeStr=boolean  PortDimensions=1
  desaturated : Inport  Port=12  OutDataTypeStr=boolean  PortDimensions=1
  spin_feasible : Inport  Port=13  OutDataTypeStr=boolean  PortDimensions=1
  spin_axis_available : Inport  Port=14  OutDataTypeStr=boolean  PortDimensions=1
  optical_target_available : Inport  Port=15  OutDataTypeStr=boolean  PortDimensions=1
  sun_sensor_valid : Inport  Port=16  OutDataTypeStr=boolean  PortDimensions=1
  intersat_sensor_tracking : Inport  Port=17  OutDataTypeStr=boolean  PortDimensions=1
  ACS_Manager : Stateflow chart  TreatAsAtomicUnit=on
      settings: PortSchema="{\"entries\":[{\"content\":{\"sides\":[{\"content\":{\"connectorIds\":[\"In2\",\"In1\",\"In3\",\"In4\",\"In5\",\"In6\",\"In7\",\"In8\",\"In9\",\"In10\",\"In11\",\"In12\",\"In13\"]},\"type\":\"ConnectorPlacement.EquallySpacedRectSide\",\"uuid\":\"c64f5ed7-7a07-4761-a251-d625087249f8\"},{\"content\":{\"connectorIds\":[\"Out1\"],\"side\":\"RIGHT\"},\"type\":\"ConnectorPlacement.EquallySpacedRectSide\",\"uuid\":\"ff17dfa7-5a32-4799-bec0-131df3b46d45\"},{\"content\":{\"side\":\"TOP\"},\"type\":\"ConnectorPlacement.EquallySpacedRectSide\",\"uuid\":\"acaf274e-12ec-4fab-ab7e-ad580afcef6e\"},{\"content\":{\"side\":\"BOTTOM\"},\"type\":\"ConnectorPlacement.EquallySpacedRectSide\",\"uuid\":\"23b8eb5a-32b2-43f2-9f21-5c184446e61f\"}]},\"type\":\"ConnectorPlacement.EquallySpacedConnector\",\"uuid\":\"7d19de63-b993-417e-b6e9-9dc888da130b\"}],\"packageUris\":[\"http://schema.mathworks.com/mf0/Connector/R2020b\"],\"version\":\"1.0\"}"
  ADS_Manager : Stateflow chart  TreatAsAtomicUnit=on
  Ephemeris_Manager : Stateflow chart  TreatAsAtomicUnit=on
      settings: PortSchema="{\"entries\":[{\"content\":{\"sides\":[{\"content\":{\"connectorIds\":[\"In2\",\"In3\",\"In1\"]},\"type\":\"ConnectorPlacement.EquallySpacedRectSide\",\"uuid\":\"cbbccf67-8c60-498d-a98a-76db8747fb3a\"},{\"content\":{\"connectorIds\":[\"Out1\"],\"side\":\"RIGHT\"},\"type\":\"ConnectorPlacement.EquallySpacedRectSide\",\"uuid\":\"743b35d2-d398-4833-9c20-93b5e77612f2\"},{\"content\":{\"side\":\"TOP\"},\"type\":\"ConnectorPlacement.EquallySpacedRectSide\",\"uuid\":\"56075cc1-c683-438a-85bf-78d94186ffa6\"}]},\"type\":\"ConnectorPlacement.EquallySpacedConnector\",\"uuid\":\"bae867d4-09fc-4097-a23b-eff5fb3633ac\"}],\"packageUris\":[\"http://schema.mathworks.com/mf0/Connector/R2020b\"],\"version\":\"1.0\"}"
  Frame_Manager : Stateflow chart  TreatAsAtomicUnit=on
  Mission_Mode_Manager : Stateflow chart  TreatAsAtomicUnit=on
  Scope : Scope
      settings: ActiveDisplayYMinimum=-1  ActiveDisplayYMaximum=1  DataLoggingVariableName=ScopeData4
  desired_ephem : Outport
  desired_ads : Outport  Port=2
  desired_frame : Outport  Port=3
  desired_acs : Outport  Port=4
  actual_ephem : Outport  Port=5
  actual_ads : Outport  Port=6
  actual_frame : Outport  Port=7
  actual_acs : Outport  Port=8
  wires:
  sun_sensor_valid/1 -> ACS_Manager/13(sun_sensor_valid)
  ACS_Manager/1(actual_acs) -> actual_acs/1
  Mission_Mode_Manager/4(desired_acs) -> Scope/1, ACS_Manager/1(desired_acs), desired_acs/1
  energy_low/1 -> ACS_Manager/6(energy_low)
  Mission_Mode_Manager/1(desired_ephem) -> Ephemeris_Manager/1(desired_ephem), desired_ephem/1
  Frame_Manager/1(actual_frame) -> actual_frame/1
  optical_target_available/1 -> ACS_Manager/12(optical_target_available)
  Mission_Mode_Manager/2(desired_ads) -> desired_ads/1, ADS_Manager/1(desired_ads)
  tle_error_high/1 -> Ephemeris_Manager/3(tle_error_high)
  reference_available/1 -> ACS_Manager/5(reference_available)
  detumbled/1 -> ACS_Manager/3(detumbled)
  wheels_saturated/1 -> ACS_Manager/8(wheels_saturated)
  Mission_Mode_Manager/3(desired_frame) -> desired_frame/1, Frame_Manager/1(desired_frame)
  ADS_Manager/1(actual_ads) -> actual_ads/1
  ads_fine_allowed/1 -> ADS_Manager/2(ads_fine_allowed)
  Ephemeris_Manager/1(actual_ephem) -> actual_ephem/1, ACS_Manager/2(actual_ephem)
  gps_valid/1 -> Ephemeris_Manager/2(gps_valid)
  intersat_sensor_tracking/1 -> Mission_Mode_Manager/2(intersat_sensor_tracking)
  ads_fault/1 -> ADS_Manager/3(ads_fault)
  recovery_ready/1 -> ACS_Manager/7(recovery_ready)
  mission_cmd/1 -> Mission_Mode_Manager/1(mission_cmd)
  spin_axis_available/1 -> ACS_Manager/11(spin_axis_available)
  desaturated/1 -> ACS_Manager/9(desaturated)
  spin_feasible/1 -> ACS_Manager/10(spin_feasible)
  zero_omega/1 -> ACS_Manager/4(zero_omega)

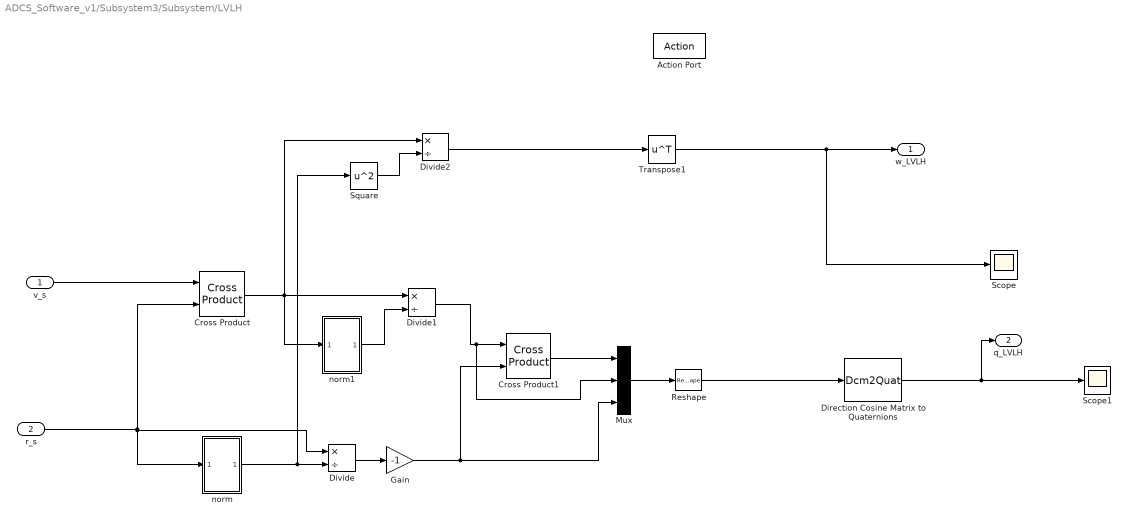
== system ADCS_Software_v1/Subsystem3/Subsystem/LVLH ==
  v_s : Inport
  r_s : Inport  Port=2
  Action Port : ActionPort  ActionPortLabel=case [ 3 ]:
  Cross Product : matrix_library/Cross Product
  Cross Product1 : matrix_library/Cross Product
  Direction Cosine Matrix to Quaternions : Dcm2Quat
  Divide : Product  Inputs=*/
  Divide1 : Product  Inputs=*/
  Divide2 : Product  Inputs=*/
  Gain : Gain  Gain=-1
  Mux : Mux  Inputs=3
  Reshape : Reshape  OutputDimensionality=Customize  OutputDimensions=[3,3]
  Scope : Scope
      settings: ActiveDisplayYMinimum=-1  ActiveDisplayYMaximum=1  DataLoggingVariableName=ScopeData6
  Scope1 : Scope
      settings: ActiveDisplayYMinimum=-0.82867069291103368  ActiveDisplayYMaximum=0.87774872275294546
  Square : Math  Operator=square
  Transpose1 : Math  Operator=transpose
  norm : Subsystem
  norm1 : Subsystem
  w_LVLH : Outport
  q_LVLH : Outport  Port=2
  wires:
  Transpose1/1 -> Scope/1, w_LVLH/1
  Divide/1 -> Gain/1
  Divide1/1 -> Mux/2, Cross Product1/1
  norm1/1(Out1) -> Divide1/2
  Cross Product1/1 -> Mux/1
  Mux/1 -> Reshape/1
  Square/1 -> Divide2/2
  v_s/1 -> Cross Product/1
  r_s/1 -> norm/1(In1), Divide/1, Cross Product/2
  norm/1(Out1) -> Square/1, Divide/2
  Divide2/1 -> Transpose1/1
  Direction Cosine Matrix to Quaternions/1 -> q_LVLH/1, Scope1/1
  Gain/1 -> Mux/3, Cross Product1/2
  Cross Product/1 -> Divide2/1, Divide1/1, norm1/1(In1)
  Reshape/1 -> Direction Cosine Matrix to Quaternions/1

== system ADCS_Software_v1/Subsystem3/Subsystem/Subsystem ==
  w2 : Inport
  q2 : Inport  Port=2
  w3 : Inport  Port=3
  q3 : Inport  Port=4
  w4 : Inport  Port=5
  q4 : Inport  Port=6
  w5 : Inport  Port=7
  q5 : Inport  Port=8
  w0 : Inport  Port=9
  q0 : Inport  Port=10
  Merge : Merge  Inputs=5
  Merge1 : Merge  Inputs=5
  Transpose2 : Math  Operator=transpose
  Out1 : Outport
  q_Ref : Outport  Port=2
  wires:
  q4/1 -> Merge1/3
  q3/1 -> Merge1/2
  Merge/1 -> Transpose2/1
  q2/1 -> Merge1/1
  Merge1/1 -> q_Ref/1
  w4/1 -> Merge/3
  w3/1 -> Merge/2
  w2/1 -> Merge/1
  Transpose2/1 -> Out1/1
  q0/1 -> Merge1/5
  q5/1 -> Merge1/4
  w0/1 -> Merge/5
  w5/1 -> Merge/4

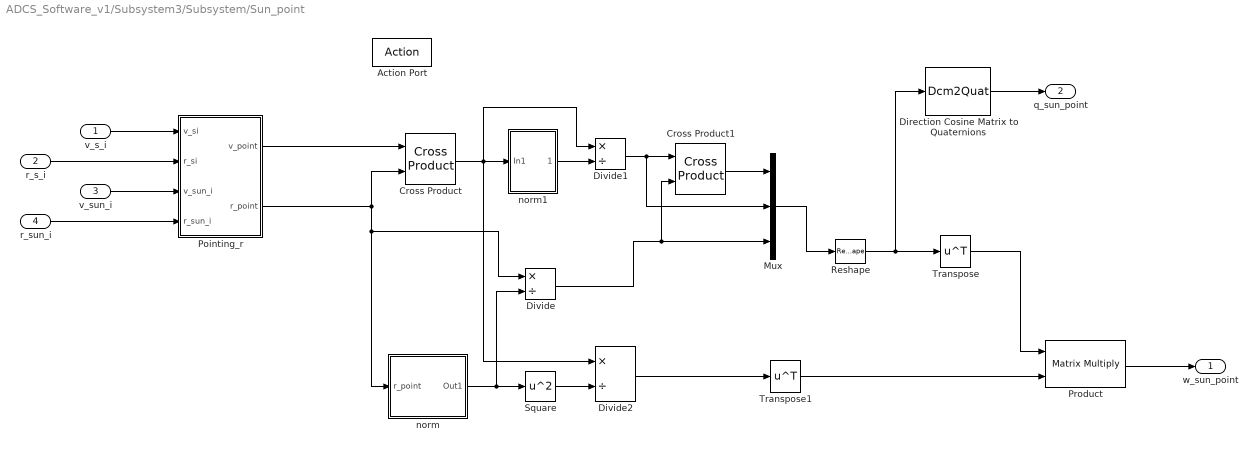
== system ADCS_Software_v1/Subsystem3/Subsystem/Sun_point ==
  v_s_i : Inport
  r_s_i : Inport  Port=2
  v_sun_i : Inport  Port=3
  r_sun_i : Inport  Port=4
  Action Port : ActionPort  ActionPortLabel=case [ 2 ]:
  Cross Product : matrix_library/Cross Product
  Cross Product1 : matrix_library/Cross Product
  Direction Cosine Matrix to Quaternions : Dcm2Quat
  Divide : Product  Inputs=*/
  Divide1 : Product  Inputs=*/
  Divide2 : Product  Inputs=*/
  Mux : Mux  Inputs=3
  Pointing_r : Subsystem
  Product : Product  Multiplication=Matrix(*)
  Reshape : Reshape  OutputDimensionality=Customize  OutputDimensions=[3,3]
  Square : Math  Operator=square
  Transpose : Math  Operator=transpose
  Transpose1 : Math  Operator=transpose
  norm : Subsystem
  norm1 : Subsystem
  w_sun_point : Outport
  q_sun_point : Outport  Port=2
  wires:
  Product/1 -> w_sun_point/1
  Direction Cosine Matrix to Quaternions/1 -> q_sun_point/1
  Transpose/1 -> Product/1
  Reshape/1 -> Transpose/1, Direction Cosine Matrix to Quaternions/1
  Transpose1/1 -> Product/2
  Cross Product1/1 -> Mux/1
  Divide/1 -> Cross Product1/2, Mux/3
  Square/1 -> Divide2/2
  norm1/1(Out1) -> Divide1/2
  Divide1/1 -> Mux/2, Cross Product1/1
  Cross Product/1 -> norm1/1(In1), Divide1/1, Divide2/1
  Pointing_r/2(r_point) -> Divide/1, norm/1(r_point), Cross Product/2
  Mux/1 -> Reshape/1
  norm/1(Out1) -> Square/1, Divide/2
  Divide2/1 -> Transpose1/1
  Pointing_r/1(v_point) -> Cross Product/1
  r_s_i/1 -> Pointing_r/2(r_si)
  v_s_i/1 -> Pointing_r/1(v_si)
  v_sun_i/1 -> Pointing_r/3(v_sun_i)
  r_sun_i/1 -> Pointing_r/4(r_sun_i)

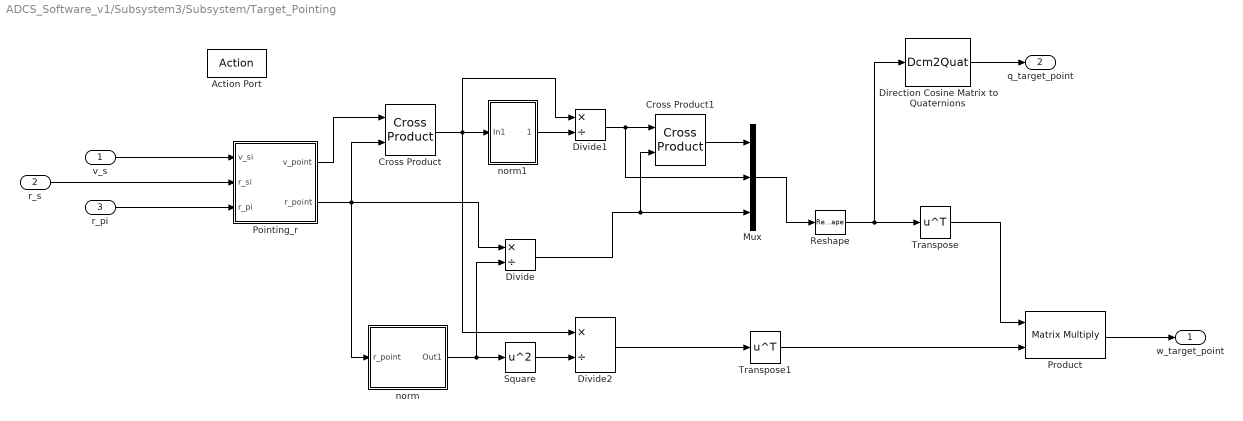
== system ADCS_Software_v1/Subsystem3/Subsystem/Target_Pointing ==
  v_s : Inport
  r_s : Inport  Port=2
  r_pi : Inport  Port=3
  Action Port : ActionPort  ActionPortLabel=case [ 4 ]:
  Cross Product : matrix_library/Cross Product
  Cross Product1 : matrix_library/Cross Product
  Direction Cosine Matrix to Quaternions : Dcm2Quat
  Divide : Product  Inputs=*/
  Divide1 : Product  Inputs=*/
  Divide2 : Product  Inputs=*/
  Mux : Mux  Inputs=3
  Pointing_r : Subsystem
  Product : Product  Multiplication=Matrix(*)
  Reshape : Reshape  OutputDimensionality=Customize  OutputDimensions=[3,3]
  Square : Math  Operator=square
  Transpose : Math  Operator=transpose
  Transpose1 : Math  Operator=transpose
  norm : Subsystem
  norm1 : Subsystem
  w_target_point : Outport
  q_target_point : Outport  Port=2
  wires:
  v_s/1 -> Pointing_r/1(v_si)
  r_s/1 -> Pointing_r/2(r_si)
  Pointing_r/1(v_point) -> Cross Product/1
  Divide2/1 -> Transpose1/1
  norm/1(Out1) -> Divide/2, Square/1
  Mux/1 -> Reshape/1
  Pointing_r/2(r_point) -> norm/1(r_point), Divide/1, Cross Product/2
  Cross Product/1 -> Divide2/1, Divide1/1, norm1/1(In1)
  Divide1/1 -> Cross Product1/1, Mux/2
  norm1/1(Out1) -> Divide1/2
  Square/1 -> Divide2/2
  Divide/1 -> Mux/3, Cross Product1/2
  Cross Product1/1 -> Mux/1
  Transpose1/1 -> Product/2
  Reshape/1 -> Direction Cosine Matrix to Quaternions/1, Transpose/1
  Transpose/1 -> Product/1
  Direction Cosine Matrix to Quaternions/1 -> q_target_point/1
  Product/1 -> w_target_point/1
  r_pi/1 -> Pointing_r/3(r_pi)

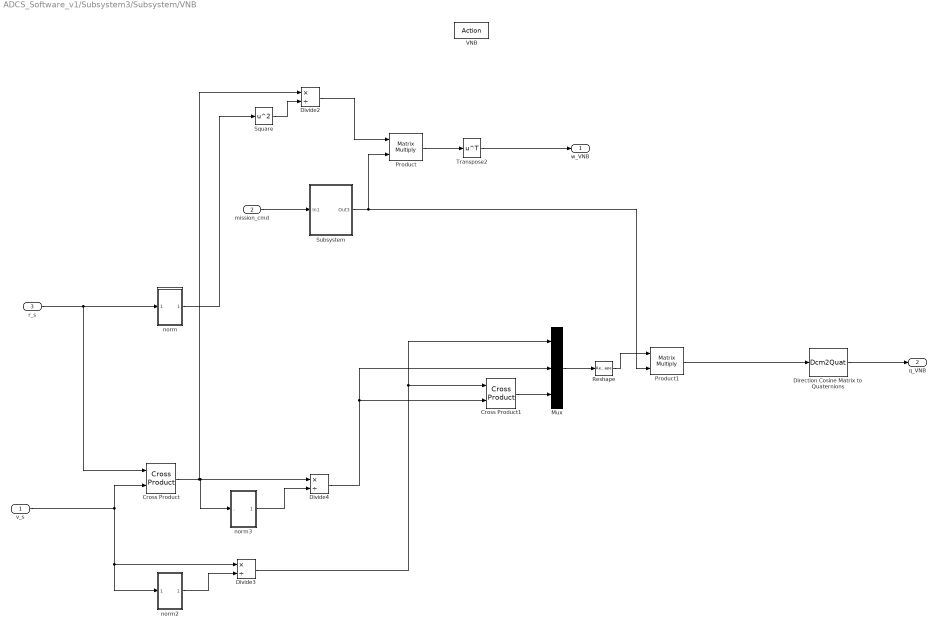
== system ADCS_Software_v1/Subsystem3/Subsystem/VNB ==
  v_s : Inport
  mission_cmd : Inport  Port=2
  r_s : Inport  Port=3
  VNB : ActionPort  ActionPortLabel=case [ 5 ]:
  Cross Product : matrix_library/Cross Product
  Cross Product1 : matrix_library/Cross Product
  Direction Cosine Matrix to Quaternions : Dcm2Quat
  Divide2 : Product  Inputs=*/
  Divide3 : Product  Inputs=*/
  Divide4 : Product  Inputs=*/
  Mux : Mux  Inputs=3
  Product : Product  Multiplication=Matrix(*)
  Product1 : Product  Multiplication=Matrix(*)
  Reshape : Reshape  OutputDimensionality=Customize  OutputDimensions=[3,3]
  Square : Math  Operator=square
  Subsystem : Subsystem
  Transpose2 : Math  Operator=transpose
  norm : Subsystem
  norm2 : Subsystem
  norm3 : Subsystem
  w_VNB : Outport
  q_VNB : Outport  Port=2
  wires:
  Product/1 -> Transpose2/1
  Square/1 -> Divide2/2
  r_s/1 -> norm/1(In1), Cross Product/1
  norm/1(Out1) -> Square/1
  Direction Cosine Matrix to Quaternions/1 -> q_VNB/1
  Product1/1 -> Direction Cosine Matrix to Quaternions/1
  norm2/1(Out1) -> Divide3/2
  v_s/1 -> Divide3/1, norm2/1(v_s), Cross Product/2
  Divide3/1 -> Mux/1, Cross Product1/1
  Cross Product/1 -> Divide2/1, norm3/1(,), Divide4/1
  norm3/1(Out1) -> Divide4/2
  Divide4/1 -> Cross Product1/2, Mux/2
  Cross Product1/1 -> Mux/3
  mission_cmd/1 -> Subsystem/1(In1)
  Subsystem/1(Out3) -> Product/2, Product1/2
  Mux/1 -> Reshape/1
  Reshape/1 -> Product1/1
  Transpose2/1 -> w_VNB/1
  Divide2/1 -> Product/1

== system ADCS_Software_v1/Subsystem3/Subsystem/default ==
  Action Port : ActionPort  ActionPortLabel=default:
  Constant : Constant  Value=[0; 0; 0]
  Constant1 : Constant  Value=[1 0 0 0]
  w_default : Outport
  q_default : Outport  Port=2
  wires:
  Constant1/1 -> q_default/1
  Constant/1 -> w_default/1

== system ADCS_Software_v1/Subsystem3/Controller/Control Algorithms/DESAT ==
  B : Inport
  RW_omega : Inport  Port=2
  desat : ActionPort  ActionPortLabel=case [ 4 ]:
  Cross Product : matrix_library/Cross Product
  Divide : Product  Inputs=*/
  Dot Product : DotProduct  OutDataTypeStr=Inherit: Inherit via internal rule
  Gain : Gain  Gain=-k_desat
  tau_cmd : Outport
  wires:
  B/1 -> Dot Product/1, Dot Product/2, Cross Product/2
  Divide/1 -> Gain/1
  Gain/1 -> tau_cmd/1
  Cross Product/1 -> Divide/1
  RW_omega/1 -> Cross Product/1
  Dot Product/1 -> Divide/2

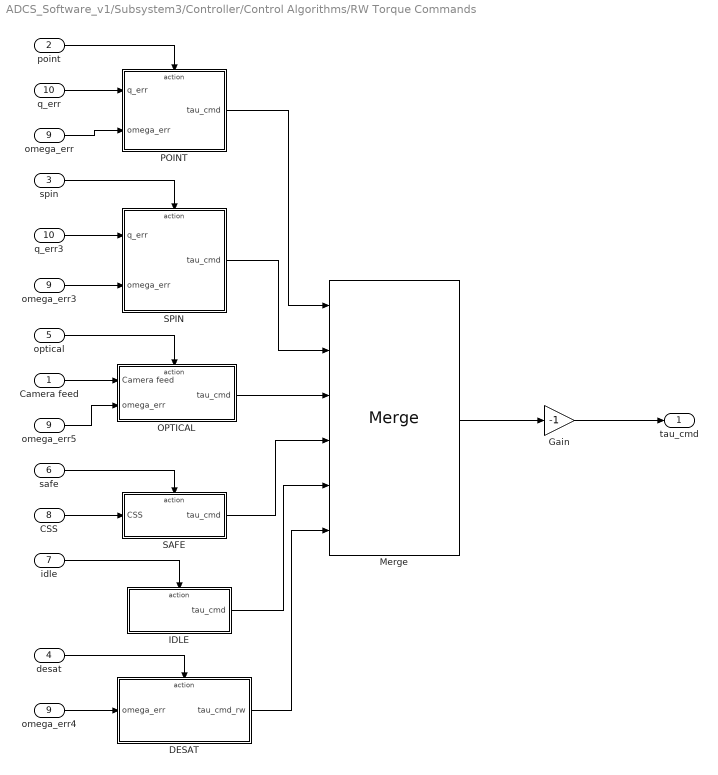
== system ADCS_Software_v1/Subsystem3/Controller/Control Algorithms/RW Torque Commands ==
  Camera feed : Inport
  point : Inport  Port=2
  spin : Inport  Port=3
  desat : Inport  Port=4
  optical : Inport  Port=5
  safe : Inport  Port=6
  idle : Inport  Port=7
  CSS : Inport  Port=8
  omega_err : Inport  Port=9
  q_err : Inport  Port=10
  DESAT : Subsystem  TreatAsAtomicUnit=on
  Gain : Gain  Gain=-1
  IDLE : Subsystem  TreatAsAtomicUnit=on
  Merge : Merge  Inputs=6
  OPTICAL : Subsystem  TreatAsAtomicUnit=on
  POINT : Subsystem  TreatAsAtomicUnit=on
  SAFE : Subsystem  TreatAsAtomicUnit=on
  SPIN : Subsystem  TreatAsAtomicUnit=on
  omega_err3 : InportShadow  Port=9
  omega_err4 : InportShadow  Port=9
  omega_err5 : InportShadow  Port=9
  q_err3 : InportShadow  Port=10
  tau_cmd : Outport
  wires:
  idle/1 -> IDLE/Action
  spin/1 -> SPIN/Action
  Camera feed/1 -> OPTICAL/1(Camera feed)
  omega_err4/1 -> DESAT/1(omega_err)
  omega_err/1 -> POINT/2(omega_err)
  optical/1 -> OPTICAL/Action
  desat/1 -> DESAT/Action
  CSS/1 -> SAFE/1(CSS)
  point/1 -> POINT/Action
  omega_err3/1 -> SPIN/2(omega_err)
  safe/1 -> SAFE/Action
  q_err/1 -> POINT/1(q_err)
  q_err3/1 -> SPIN/1(q_err)
  omega_err5/1 -> OPTICAL/2(omega_err)
  POINT/1(tau_cmd) -> Merge/1
  SPIN/1(tau_cmd) -> Merge/2
  OPTICAL/1(tau_cmd) -> Merge/3
  SAFE/1(tau_cmd) -> Merge/4
  IDLE/1(tau_cmd) -> Merge/5
  DESAT/1(tau_cmd_rw) -> Merge/6
  Merge/1 -> Gain/1
  Gain/1 -> tau_cmd/1

== system ADCS_Software_v1/Subsystem3/Controller/Control Algorithms/Thruster Torque commands ==
  detumble : Inport
  desat : Inport  Port=2
  default : Inport  Port=3
  omega : Inport  Port=4
  RW_omega : Inport  Port=5
  DEFAULT : Subsystem  TreatAsAtomicUnit=on
  DESAT : Subsystem  TreatAsAtomicUnit=on
  DETUMBLE : Subsystem  TreatAsAtomicUnit=on
  Merge1 : Merge  Inputs=3
  tau_cmd : Outport
  wires:
  omega/1 -> DETUMBLE/1(omega)
  DETUMBLE/1(tau_cmd) -> Merge1/1
  Merge1/1 -> tau_cmd/1
  detumble/1 -> DETUMBLE/Action
  default/1 -> DEFAULT/Action
  DEFAULT/1(tau_cmd) -> Merge1/3
  RW_omega/1 -> DESAT/1(RW_omega)
  desat/1 -> DESAT/Action
  DESAT/1(tau_cmd) -> Merge1/2

== system ADCS_Software_v1/Subsystem3/Controller/Control Algorithms/default ==
  detumble : ActionPort  ActionPortLabel=default:
  Constant : Constant  Value=[0 0 0]
  tau_cmd : Outport
  wires:
  Constant/1 -> tau_cmd/1

== system ADCS_Software_v1/Subsystem3/Subsystem/LVLH/norm ==
  In1 : Inport
  Sqrt : Sqrt
  Square : Math  Operator=square
  Sum of Elements : Sum  Inputs=+
  Out1 : Outport
  wires:
  In1/1 -> Square/1
  Square/1 -> Sum of Elements/1
  Sum of Elements/1 -> Sqrt/1
  Sqrt/1 -> Out1/1

== system ADCS_Software_v1/Subsystem3/Subsystem/LVLH/norm1 ==
  In1 : Inport
  Sqrt : Sqrt
  Square : Math  Operator=square
  Sum of Elements : Sum  Inputs=+
  Out1 : Outport
  wires:
  Sqrt/1 -> Out1/1
  Sum of Elements/1 -> Sqrt/1
  Square/1 -> Sum of Elements/1
  In1/1 -> Square/1

== system ADCS_Software_v1/Subsystem3/Subsystem/Sun_point/Pointing_r ==
  v_si : Inport
  r_si : Inport  Port=2
  v_sun_i : Inport  Port=3
  r_sun_i : Inport  Port=4
  Sum : Sum  Inputs=|-+
  Sum1 : Sum  Inputs=|-+
  v_point : Outport
  r_point : Outport  Port=2
  wires:
  Sum1/1 -> v_point/1
  v_si/1 -> Sum1/1
  Sum/1 -> r_point/1
  r_si/1 -> Sum/1
  v_sun_i/1 -> Sum1/2
  r_sun_i/1 -> Sum/2

== system ADCS_Software_v1/Subsystem3/Subsystem/Sun_point/norm ==
  r_point : Inport
  Sqrt : Sqrt
  Square : Math  Operator=square
  Sum of Elements : Sum  Inputs=+
  Out1 : Outport
  wires:
  r_point/1 -> Square/1
  Square/1 -> Sum of Elements/1
  Sum of Elements/1 -> Sqrt/1
  Sqrt/1 -> Out1/1

== system ADCS_Software_v1/Subsystem3/Subsystem/Sun_point/norm1 ==
  In1 : Inport
  Sqrt : Sqrt
  Square : Math  Operator=square
  Sum of Elements : Sum  Inputs=+
  Out1 : Outport
  wires:
  Sqrt/1 -> Out1/1
  Sum of Elements/1 -> Sqrt/1
  Square/1 -> Sum of Elements/1
  In1/1 -> Square/1

== system ADCS_Software_v1/Subsystem3/Subsystem/Target_Pointing/Pointing_r ==
  v_si : Inport
  r_si : Inport  Port=2
  r_pi : Inport  Port=3
  Sum : Sum  Inputs=-+|
  Sum1 : Sum  Inputs=|-+
  omega_E : Constant  Value=[0 0 7.2921159e-5]
  v_p : matrix_library/Cross Product
  v_point : Outport
  r_point : Outport  Port=2
  wires:
  r_si/1 -> Sum/1
  r_pi/1 -> v_p/2, Sum/2
  Sum/1 -> r_point/1
  v_si/1 -> Sum1/1
  omega_E/1 -> v_p/1
  Sum1/1 -> v_point/1
  v_p/1 -> Sum1/2

== system ADCS_Software_v1/Subsystem3/Subsystem/Target_Pointing/norm ==
  r_point : Inport
  Sqrt : Sqrt
  Square : Math  Operator=square
  Sum of Elements : Sum  Inputs=+
  Out1 : Outport
  wires:
  Sqrt/1 -> Out1/1
  Sum of Elements/1 -> Sqrt/1
  Square/1 -> Sum of Elements/1
  r_point/1 -> Square/1

== system ADCS_Software_v1/Subsystem3/Subsystem/Target_Pointing/norm1 ==
  In1 : Inport
  Sqrt : Sqrt
  Square : Math  Operator=square
  Sum of Elements : Sum  Inputs=+
  Out1 : Outport
  wires:
  In1/1 -> Square/1
  Square/1 -> Sum of Elements/1
  Sum of Elements/1 -> Sqrt/1
  Sqrt/1 -> Out1/1

== system ADCS_Software_v1/Subsystem3/Subsystem/VNB/Subsystem ==
  In1 : Inport
  Default : Subsystem  TreatAsAtomicUnit=on
  M_MAX_DRAG : Subsystem  TreatAsAtomicUnit=on
  M_MIN_DRAG : Subsystem  TreatAsAtomicUnit=on
  M_RAM : Subsystem  TreatAsAtomicUnit=on
  Merge : Merge  Inputs=4
  Switch Case : SwitchCase  CaseConditions={8,9,10}
  Out3 : Outport
  wires:
  Switch Case/1 -> M_MIN_DRAG/Action
  In1/1 -> Switch Case/1
  Switch Case/4 -> Default/Action
  Switch Case/3 -> M_RAM/Action
  Switch Case/2 -> M_MAX_DRAG/Action
  Merge/1 -> Out3/1
  M_MIN_DRAG/1(Out1) -> Merge/1
  M_MAX_DRAG/1(Out1) -> Merge/2
  M_RAM/1(Out1) -> Merge/3
  Default/1(Out1) -> Merge/4

== system ADCS_Software_v1/Subsystem3/Subsystem/VNB/norm ==
  In1 : Inport
  Sqrt : Sqrt
  Square : Math  Operator=square
  Sum of Elements : Sum  Inputs=+
  Out1 : Outport
  wires:
  In1/1 -> Square/1
  Square/1 -> Sum of Elements/1
  Sum of Elements/1 -> Sqrt/1
  Sqrt/1 -> Out1/1

== system ADCS_Software_v1/Subsystem3/Subsystem/VNB/norm2 ==
  v_s : Inport
  Sqrt : Sqrt
  Square : Math  Operator=square
  Sum of Elements : Sum  Inputs=+
  Out1 : Outport
  wires:
  Sqrt/1 -> Out1/1
  Sum of Elements/1 -> Sqrt/1
  Square/1 -> Sum of Elements/1
  v_s/1 -> Square/1

== system ADCS_Software_v1/Subsystem3/Subsystem/VNB/norm3 ==
  , : Inport
  Sqrt : Sqrt
  Square : Math  Operator=square
  Sum of Elements : Sum  Inputs=+
  Out1 : Outport
  wires:
  Sqrt/1 -> Out1/1
  Sum of Elements/1 -> Sqrt/1
  Square/1 -> Sum of Elements/1
  ,/1 -> Square/1

== system ADCS_Software_v1/Subsystem3/Controller/Control Algorithms/RW Torque Commands/DESAT ==
  omega_err : Inport
  desat : ActionPort  ActionPortLabel=case [ 4 ]:
  Gain1 : Gain  Gain=-kd_point
  tau_cmd_rw : Outport
  wires:
  omega_err/1 -> Gain1/1
  Gain1/1 -> tau_cmd_rw/1

== system ADCS_Software_v1/Subsystem3/Controller/Control Algorithms/RW Torque Commands/IDLE ==
  idle : ActionPort  ActionPortLabel=default:
  Constant : Constant  Value=[0 0 0]
  tau_cmd : Outport
  wires:
  Constant/1 -> tau_cmd/1

== system ADCS_Software_v1/Subsystem3/Controller/Control Algorithms/RW Torque Commands/OPTICAL ==
  Camera feed : Inport
  omega_err : Inport  Port=2
  optical : ActionPort  ActionPortLabel=case [ 5 ]:
  Constant1 : Constant  Value=0
  Gain1 : Gain  Gain=kd_point
  Gain2 : Gain  Gain=kp_point*0.005
  Gain3 : Gain  Gain=-1
  MATLAB Function2 : MATLAB Function  TreatAsAtomicUnit=on
  Mux : Mux  Inputs=3
  Sum1 : Sum  Inputs=|+-
  tau_cmd : Outport
  wires:
  Camera feed/1 -> MATLAB Function2/1(u)
  Gain1/1 -> Sum1/2
  Sum1/1 -> tau_cmd/1
  Mux/1 -> Gain2/1
  Gain2/1 -> Sum1/1
  Constant1/1 -> Mux/3
  MATLAB Function2/2(x_cm) -> Mux/2
  omega_err/1 -> Gain1/1
  MATLAB Function2/1(y_cm) -> Gain3/1
  Gain3/1 -> Mux/1

== system ADCS_Software_v1/Subsystem3/Controller/Control Algorithms/RW Torque Commands/POINT ==
  q_err : Inport
  omega_err : Inport  Port=2
  point : ActionPort  ActionPortLabel=case [ 2 ]:
  Gain : Gain  Gain=-kd_point
  Gain1 : Gain  Gain=kp_point
  Sum : Sum  Inputs=|++
  tau_cmd : Outport
  wires:
  Sum/1 -> tau_cmd/1
  omega_err/1 -> Gain/1
  Gain1/1 -> Sum/1
  Gain/1 -> Sum/2
  q_err/1 -> Gain1/1

== system ADCS_Software_v1/Subsystem3/Controller/Control Algorithms/RW Torque Commands/SAFE ==
  CSS : Inport
  safe : ActionPort  ActionPortLabel=case [ 6 ]:
  Constant : Constant  Value=[0 0 0]
  tau_cmd : Outport
  wires:
  Constant/1 -> tau_cmd/1

== system ADCS_Software_v1/Subsystem3/Controller/Control Algorithms/RW Torque Commands/SPIN ==
  q_err : Inport
  omega_err : Inport  Port=2
  spin : ActionPort  ActionPortLabel=case [ 3 ]:
  Constant : Constant  Value=[0 0 1]
  Constant1 : Constant  Value=[1 1 1]
  Gain : Gain  Gain=kd_spin
  Gain1 : Gain  Gain=kp_spin
  Gain2 : Gain  Gain=0.04
  Product : Product
  Sum : Sum  Inputs=|+-
  Sum1 : Sum  Inputs=|+-
  Sum2 : Sum  Inputs=|+-
  tau_cmd : Outport
  wires:
  Sum/1 -> Gain/1
  omega_err/1 -> Sum/1
  Constant/1 -> Sum2/2, Gain2/1
  Gain/1 -> Sum1/2
  Sum1/1 -> tau_cmd/1
  Constant1/1 -> Sum2/1
  q_err/1 -> Product/1
  Sum2/1 -> Product/2
  Product/1 -> Gain1/1
  Gain1/1 -> Sum1/1
  Gain2/1 -> Sum/2

== system ADCS_Software_v1/Subsystem3/Controller/Control Algorithms/Thruster Torque commands/DEFAULT ==
  default : ActionPort  ActionPortLabel=default:
  Constant : Constant  Value=[0 0 0]
  tau_cmd : Outport
  wires:
  Constant/1 -> tau_cmd/1

== system ADCS_Software_v1/Subsystem3/Controller/Control Algorithms/Thruster Torque commands/DESAT ==
  RW_omega : Inport
  desat : ActionPort  ActionPortLabel=case [ 4 ]:
  Gain2 : Gain  Gain=-k_desat
  tau_cmd : Outport
  wires:
  RW_omega/1 -> Gain2/1
  Gain2/1 -> tau_cmd/1

== system ADCS_Software_v1/Subsystem3/Controller/Control Algorithms/Thruster Torque commands/DETUMBLE ==
  omega : Inport
  detumble : ActionPort  ActionPortLabel=case [ 1 ]:
  Gain : Gain  Gain=-kd_detumble
  tau_cmd : Outport
  wires:
  omega/1 -> Gain/1
  Gain/1 -> tau_cmd/1

== system ADCS_Software_v1/Subsystem3/Subsystem/VNB/Subsystem/Default ==
  min drag : ActionPort  ActionPortLabel=default:
  Constant : Constant  Value=[1 0 0; 0 1 0; 0 0 1]
  Out1 : Outport
  wires:
  Constant/1 -> Out1/1

== system ADCS_Software_v1/Subsystem3/Subsystem/VNB/Subsystem/M_MAX_DRAG ==
  max drag : ActionPort  ActionPortLabel=case [ 9 ]:
  Constant : Constant  Value=[0 0 1; 0 1 0; -1 0 0]
  Out1 : Outport
  wires:
  Constant/1 -> Out1/1

== system ADCS_Software_v1/Subsystem3/Subsystem/VNB/Subsystem/M_MIN_DRAG ==
  min drag : ActionPort  ActionPortLabel=case [ 8 ]:
  Constant : Constant  Value=[1 0 0; 0 1 0; 0 0 1]
  Out1 : Outport
  wires:
  Constant/1 -> Out1/1

== system ADCS_Software_v1/Subsystem3/Subsystem/VNB/Subsystem/M_RAM ==
  RAM : ActionPort  ActionPortLabel=case [ 10 ]:
  Constant1 : Constant  Value=[0 0 1; 0 1 0; -1 0 0]
  Out1 : Outport
  wires:
  Constant1/1 -> Out1/1

== stateflow chart ADCS_Software_v1/Subsystem3/Mode manager/Mode Manager/Frame_Manager ==
  state FRAME_INERTIAL
    entry:
    actual_frame = uint8(2);
  state FRAME_LVLH
    entry:
    actual_frame = uint8(3);
  state FRAME_BODY
    entry:
    actual_frame = uint8(1);
  state FRAME_EARTH_TARGET
    entry:
    actual_frame = uint8(4);
  state FRAME_IDLE
    entry:
    actual_frame = uint8(0);
  state FRAME_IMAGING_TDI
    entry:
    actual_frame = uint8(6);
  state FRAME_VNB
    entry:
    actual_frame = uint8(5);
  FRAME_INERTIAL -> (junction 11) : [desired_frame ~= uint8(2)]
  (junction 11) -> FRAME_INERTIAL [order 3] : [desired_frame == uint8(2)]
  FRAME_LVLH -> (junction 11) : [desired_frame ~= uint8(3)]
  (junction 11) -> FRAME_LVLH [order 4] : [desired_frame == uint8(3)]
  FRAME_BODY -> (junction 11) : [desired_frame ~= uint8(1)]
  (junction 11) -> FRAME_BODY [order 2] : [desired_frame == uint8(1)]
  FRAME_EARTH_TARGET -> (junction 11) : [desired_frame ~= uint8(4)]
  (junction 11) -> FRAME_EARTH_TARGET [order 5] : [desired_frame == uint8(4)]
  (junction 11) -> FRAME_IDLE [order 1] : [desired_frame == uint8(0)]
  FRAME_IDLE -> (junction 11) : [desired_frame ~= uint8(0)]
  FRAME_IMAGING_TDI -> (junction 11) : [desired_frame ~= uint8(6)]
  (junction 11) -> FRAME_VNB [order 6] : [desired_frame == uint8(5)]
  (junction 11) -> FRAME_IMAGING_TDI [order 7] : [desired_frame == uint8(6)]
  FRAME_VNB -> (junction 11) : [desired_frame ~= uint8(5)]
  (default) -> FRAME_IDLE
  data: desired_frame input uint8; actual_frame output uint8 =0

== stateflow chart ADCS_Software_v1/Subsystem3/Mode manager/Mode Manager/ACS_Manager ==
  state ACS_DETUMBLE
    entry:
    actual_acs = uint8(1);
    exit:
    if desired_acs == uint8(1)
    desired_acs == uint8(0)
    end
  state ACS_POINT
    entry:
    actual_acs = uint8(2);
  state ACS_IDLE
    entry:
    actual_acs = uint8(0);
  state ACS_DESAT
    entry:
    actual_acs = uint8(4);
    exit:
    if desired_acs == uint8(4)
    desired_acs == uint8(0)
    end
  state ACS_OPTICAL
    entry:
    actual_acs = uint8(5);
  state ACS_SPIN
    entry:
    actual_acs = uint8(3);
  state ACS_SAFE
    entry:
    actual_acs = uint8(6);
  ACS_OPTICAL -> ACS_POINT [order 3] : [~optical_target_available &&...
      |  ~energy_low]
  (junction 25) -> ACS_DETUMBLE [order 2] : [(desired_acs == uint8(1)&&desaturated)  ...
      | ||~detumbled]
  ACS_DETUMBLE -> (junction 25) : [ zero_omega]
  ACS_POINT -> ACS_SAFE [order 2] : [energy_low || ~reference_available ||...
      |  actual_ephem == uint8(0)]%~detumbled ||
  ACS_POINT -> (junction 25) [order 1] : [desired_acs ~= uint8(2) ||...
      | ~detumbled]
  (junction 25) -> ACS_POINT [order 3] : [desired_acs == uint8(2) && detumbled && desaturated]
  (default) -> ACS_IDLE
  (junction 25) -> ACS_IDLE [order 1] : [desired_acs == uint8(0) && detumbled && desaturated]
  ACS_IDLE -> (junction 25) : [desired_acs ~= uint8(0)]
  ACS_DESAT -> (junction 25) [order 1] : [desaturated ]%&& recovery_ready &&~energy_low
  (junction 25) -> ACS_DESAT [order 5] : [desired_acs == uint8(4)||wheels_saturated]
  (junction 25) -> ACS_OPTICAL [order 6] : [desired_acs == uint8(5)]
  ACS_OPTICAL -> (junction 25) [order 1] : [desired_acs ~= uint8(5) && optical_target_available]
  ACS_SAFE -> (junction 25) : [desired_acs ~= uint8(9) &&...
      |  ~energy_low && recovery_ready &&...
      |  sun_sensor_valid && ~((desired_acs == uint8(2)) &&...
      |  ~reference_available) && ~((desired_acs == uint8(6)) &&...
      |  (~spin_feasible || ~spin_axis_available))]
  (junction 25) -> ACS_SAFE [order 7] : [desired_acs == uint8(9)]
  (junction 25) -> ACS_SPIN [order 4] : [desired_acs == uint8(3)]
  ACS_SPIN -> (junction 25) [order 2] : [desired_acs ~= uint8(3)]
  ACS_DESAT -> ACS_SAFE [order 2] : [energy_low]
  ACS_OPTICAL -> ACS_SAFE [order 2] : [energy_low]
  ACS_SPIN -> ACS_SAFE [order 1] : [energy_low || ~spin_feasible ||...
      |  ~spin_axis_available]
  data: desired_acs input uint8; actual_ephem input uint8; detumbled input boolean; zero_omega input; reference_available input boolean; energy_low input boolean; recovery_ready input boolean; wheels_saturated input boolean; desaturated input boolean; spin_feasible input boolean; spin_axis_available input boolean; optical_target_available input boolean; sun_sensor_valid input boolean; actual_acs output uint8 =0
